simulink model "winddd"  (R2025a)
settings: Solver=ode23s  StartTime=0.0  StopTime=10.0  RelTol=1e-3
libraries: simulink x1
settings Model: Creator=Rishitha  LastModifiedBy=Rishitha

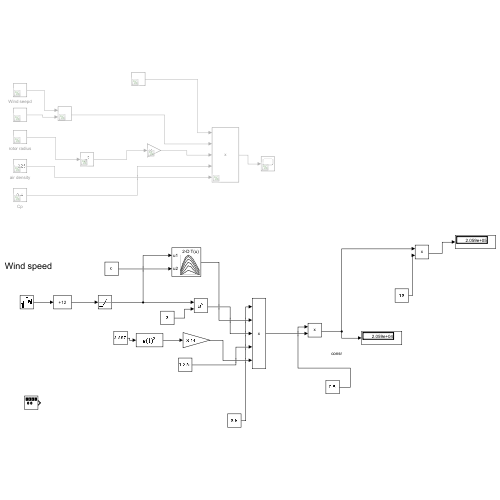
[thumbnail: Simulink's stored preview of the top-level diagram]
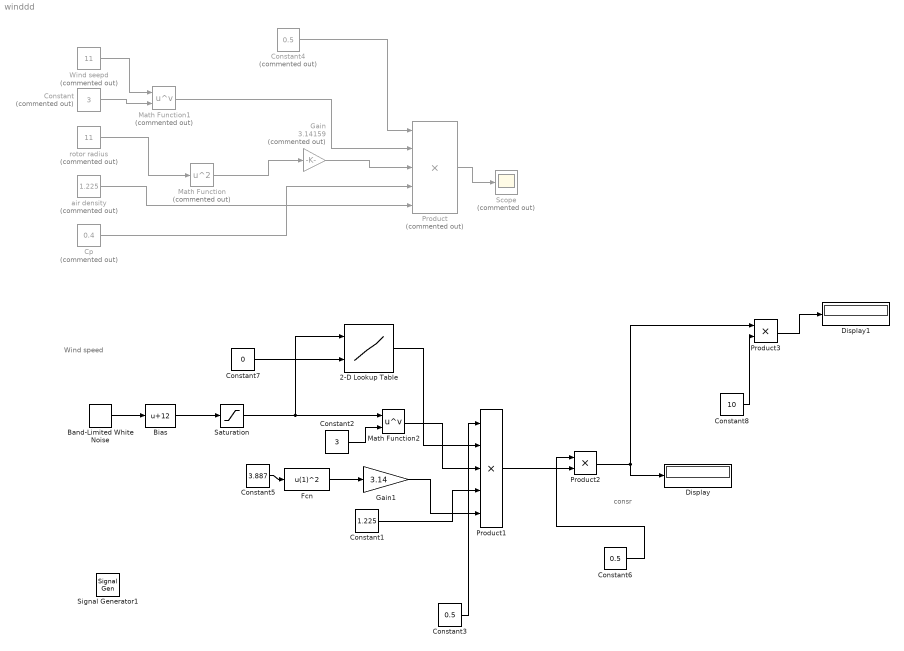
== system winddd ==
  note: consr
  note: Wind speed
  2-D Lookup Table : Lookup_n-D  BreakpointsForDimension1=[3 6 9 12 15 18 21 25]  BreakpointsForDimension2=[0 5 10 15 20 25]  Table=|  InternalRulePriority=Speed  RndMeth=Simplest
      | [0.10 0.08 0.05 0.03 0.01 0.00;
      |  0.25 0.20 0.15 0.10 0.05 0.02;
      |  0.40 0.35 0.28 0.20 0.12 0.06;
      |  0.45 0.42 0.35 0.28 0.20 0.10;
      |  0.42 0.38 0.32 0.25 0.18 0.08;
      |  0.35 0.30 0.25 0.18 0.12 0.06;
      |  0.25 0.20 0.15 0.10 0.06 0.03;
      |  0.10 0.08 0.05 0.03 0.01 0.00]
      settings: InputPortMap=u0,u1
  Band-Limited White Noise : simulink/Sources/Band-Limited White Noise  Cov=1  Ts=0.1  seed=[23341]
  Bias : Bias  Bias=12  SaturateOnIntegerOverflow=off
  Constant : Constant  Commented=on  Value=3
  Constant1 : Constant  Value=1.225
  Constant2 : Constant  Value=3
  Constant3 : Constant  Value=0.5
  Constant4 : Constant  Commented=on  Value=0.5
  Constant5 : Constant  Value=3.887
  Constant6 : Constant  Value=0.5
  Constant7 : Constant  Value=0
  Constant8 : Constant  Value=10
  Cp : Constant  Commented=on  Value=0.4
  Display : Display
  Display1 : Display
  Fcn : Fcn  Expr=u(1)^2
  Gain : Gain  Commented=on  Gain=3.14159
  Gain1 : Gain  Gain=3.14
  Math Function : Math  Commented=on  Operator=square
  Math Function1 : Math  Commented=on  Operator=pow
  Math Function2 : Math  Operator=pow
  Product : Product  Commented=on  Inputs=5
  Product1 : Product  Inputs=5
  Product2 : Product
  Product3 : Product
  Saturation : Saturate  UpperLimit=15  LowerLimit=5
  Scope : Scope  Commented=on
      settings: ActiveDisplayYMinimum=23959.271717050011  ActiveDisplayYMaximum=223959.27171705
  Signal Generator1 : SignalGenerator  Amplitude=0.5  Frequency=0.05  Units=rad/sec
  Wind seepd : Constant  Commented=on  Value=11
  air density : Constant  Commented=on  Value=1.225
  rotor radius : Constant  Commented=on  Value=11
  wires:
  Math Function/1 -> Gain/1
  Constant4/1 -> Product/1
  Math Function1/1 -> Product/2
  Gain/1 -> Product/3
  Cp/1 -> Product/4
  rotor radius/1 -> Math Function/1
  Wind seepd/1 -> Math Function1/1
  Constant/1 -> Math Function1/2
  air density/1 -> Product/5
  Product/1 -> Scope/1
  Band-Limited White Noise/1 -> Bias/1
  Bias/1 -> Saturation/1
  Saturation/1 -> 2-D Lookup Table/1, Math Function2/1
  Constant2/1 -> Math Function2/2
  Constant3/1 -> Product1/1
  2-D Lookup Table/1 -> Product1/2
  Math Function2/1 -> Product1/3
  Constant1/1 -> Product1/4
  Constant7/1 -> 2-D Lookup Table/2
  Constant5/1 -> Fcn/1
  Fcn/1 -> Gain1/1
  Gain1/1 -> Product1/5
  Product1/1 -> Product2/2
  Constant6/1 -> Product2/1
  Product2/1 -> Display/1, Product3/1
  Constant8/1 -> Product3/2
  Product3/1 -> Display1/1
